simulink subsystem "FromOmega2toThrust"  (R2026a)
settings: Solver=VariableStepAuto
undefined symbols (not defined in the file): HexaConstants
settings Model: Creator=Dell  LastModifiedBy=Carlos Fabian

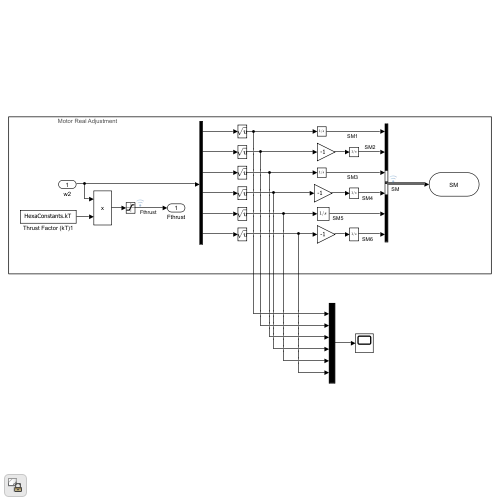
[thumbnail: Simulink's stored preview of the top-level diagram]
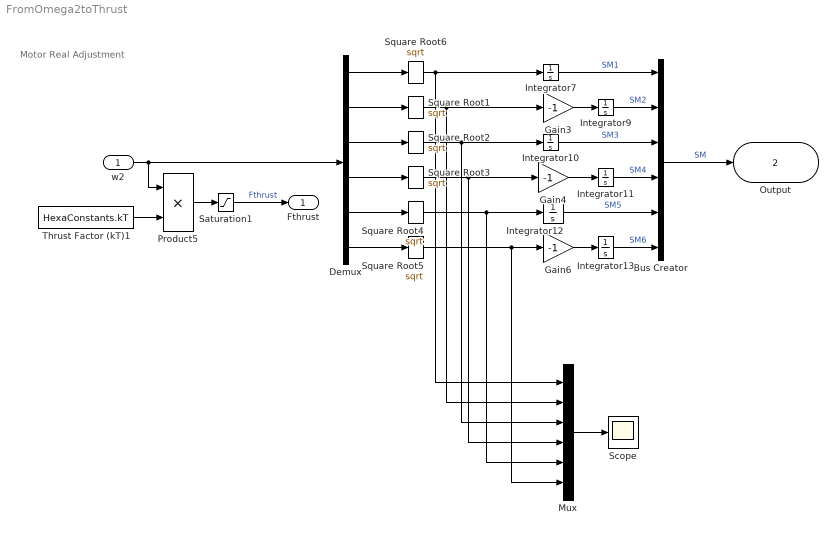
== system FromOmega2toThrust ==
  note: Motor Real Adjustment
  w2 : Inport
  Bus Creator : BusCreator  Inputs=6
  Demux : Demux  Outputs=6
  Gain3 : Gain  Gain=-1
  Gain4 : Gain  Gain=-1
  Gain6 : Gain  Gain=-1
  Integrator{7,9..13} (6 alike) : Integrator
  Mux : Mux  Inputs=6
  Product5 : Product
  Saturation1 : Saturate  UpperLimit=7  LowerLimit=0
  Scope : Scope
      settings: ActiveDisplayYMinimum=568.53095899492769  ActiveDisplayYMaximum=706.56292736040791
  Square Root{1..6} (6 alike) : Sqrt
  Thrust Factor (kT)1 : Constant  Value=HexaConstants.kT
  Fthrust : Outport
  Output : Outport  Port=2
  wires:
  Product5/1 -> Saturation1/1
  Thrust Factor (kT)1/1 -> Product5/2
  Saturation1/1 -> Fthrust/1  "Fthrust"
  w2/1 -> Product5/1, Demux/1
  Demux/2 -> Square Root1/1
  Bus Creator/1 -> Output/1  "SM"
  Demux/3 -> Square Root2/1
  Gain4/1 -> Integrator11/1
  Integrator13/1 -> Bus Creator/6  "SM6"
  Integrator10/1 -> Bus Creator/3  "SM3"
  Gain6/1 -> Integrator13/1
  Gain3/1 -> Integrator9/1
  Integrator11/1 -> Bus Creator/4  "SM4"
  Demux/6 -> Square Root5/1
  Integrator7/1 -> Bus Creator/1  "SM1"
  Demux/5 -> Square Root4/1
  Demux/4 -> Square Root3/1
  Integrator9/1 -> Bus Creator/2  "SM2"
  Integrator12/1 -> Bus Creator/5  "SM5"
  Demux/1 -> Square Root6/1
  Square Root1/1 -> Gain3/1, Mux/2
  Square Root2/1 -> Integrator10/1, Mux/3
  Square Root3/1 -> Gain4/1, Mux/4
  Square Root4/1 -> Integrator12/1, Mux/5
  Square Root5/1 -> Gain6/1, Mux/6
  Mux/1 -> Scope/1
  Square Root6/1 -> Integrator7/1, Mux/1
